simulink model "DCDC_PSFB_with_Mosfet_Converter"  (R2024b)
settings: Solver=ode23t  StartTime=0.0  StopTime=0.2  RelTol=1e-3
values from neighbouring files (symbols this model uses):
  fs = 140e3    (= 140000)    [PSFB_Calculation_Code.m]    (also in PSFB_DCDC_Conveter_Calculation.m)
  Pout = 5500    [PSFB_Calculation_Code.m]    (also in PSFB_DCDC_Conveter_Calculation.m)
  R_load = (Vout^2) / Pout    (= 116.363636364)    [PSFB_Calculation_Code.m]    (also in PSFB_DCDC_Conveter_Calculation.m = 0.104727272727)
  Ts = 1/fs    (= 7.14285714286e-06)    [PSFB_Calculation_Code.m]    (also in PSFB_DCDC_Conveter_Calculation.m)
  Vin = 24    [PSFB_Calculation_Code.m]    (also in PSFB_DCDC_Conveter_Calculation.m = 800)
  Vout = 800    [PSFB_Calculation_Code.m]    (also in PSFB_DCDC_Conveter_Calculation.m = 24; PSFB_Result_Plot_Code.m = Vout_sig.Data(:))
  Vout_max = 815    [PSFB_Calculation_Code.m]    (also in PSFB_DCDC_Conveter_Calculation.m = 25)
undefined symbols (not defined in the file or in its folder): C, L
libraries: spsMosfetLib x8, spsCurrentMeasurementLib x6, spsSeriesRLCBranchLib x6, spsDiodeLib x4, spsVoltageMeasurementLib x4, spsMeanLib x3, slpidlib x2, spsDCVoltageSourceLib x1, spsGroundLib x1, spsLinearTransformerLib x1, sps_lib x1
settings Model: Creator=SUDHAK1  LastModifiedBy=SUDHAK1

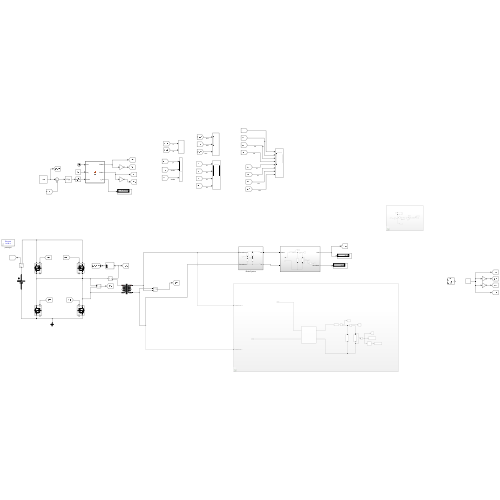
[thumbnail: Simulink's stored preview of the top-level diagram]
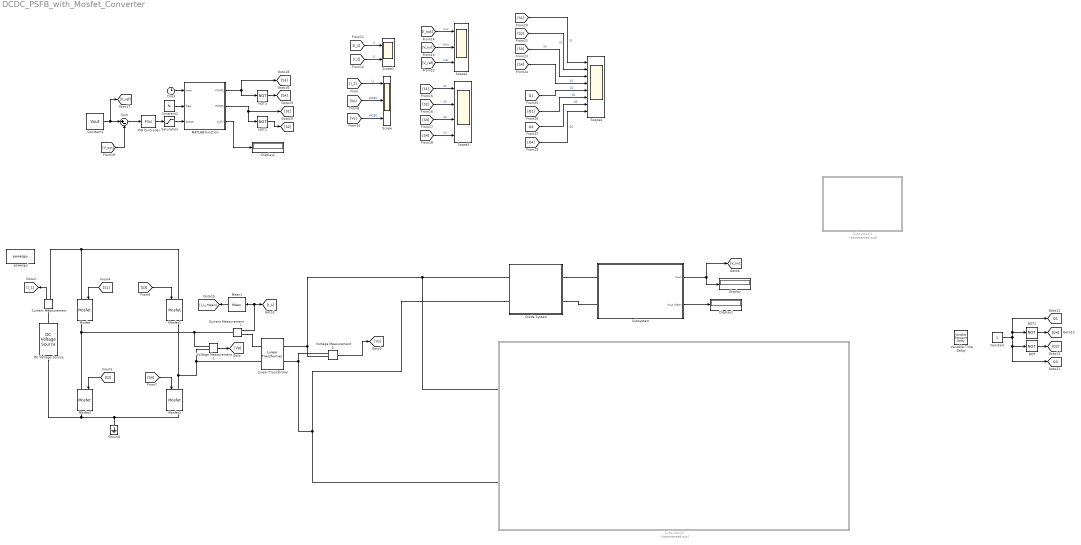
== system DCDC_PSFB_with_Mosfet_Converter ==
  Clock : Clock
  Constant : Constant
  Constant1 : Constant  Value=Vout
  Constant2 : Constant  Value=fs
  Current Measurement : spsCurrentMeasurementLib/Current Measurement  PhasorSimulation=off  OutputType=Complex  PSBequivalent=0
  Current Measurement1 : spsCurrentMeasurementLib/Current Measurement  PhasorSimulation=off  OutputType=Complex  PSBequivalent=0
  DC Voltage Source : spsDCVoltageSourceLib/DC Voltage Source  Amplitude=Vin  Measurements=None
  Diode System : Subsystem
  Display : Display
  Display1 : Display
  Display2 : Display
  Ground : spsGroundLib/Ground  LConnTagsString=a
  Linear Transformer : spsLinearTransformerLib/Linear Transformer  UNITS=SI  NominalPower=[Pout fs]  winding1=[Vin 4.3218e-9 0.45856e-9]  winding2=[Vout_max 0.7938e-9 0.084225e-9]  ThreeWindings=off  winding3=[Vout_max 0.7938e-9 0.084225e-9]  RmLm=[1.0804e+06 2866]  Measurements=None  DataType=on
  MATLAB Function : MATLAB Function  TreatAsAtomicUnit=on
  Mean1 : spsMeanLib/Mean  Freq=60  Vinit=0  Ts=0
  Mosfet{,1..3} (4 alike) : spsMosfetLib/Mosfet  Ron=0.1  Lon=0  Rd=0.01  Vfd=0  IC=0  Rs=1e5  Cs=inf  Measurements=on
  NOT{,1..3} (4 alike) : Logic  Operator=NOT  IconShape=distinctive  AllPortsSameDT=off  OutDataTypeStr=boolean
  PID Controller : slpidlib/PID Controller  Controller=PI  Form=Parallel  TimeDomain=Discrete-time  UseExternalTs=off  SampleTime=-1  IntegratorMethod=Forward Euler  FilterMethod=Forward Euler  ControllerParametersSource=internal  P=500  I=50  UseKiTs=off  D=0  UseExternalDerivativeSource=off  N=100  UseFilter=on  TunerSelectOption=Transfer Function Based (PID Tuner App)  InitialConditionSource=internal  InitialConditionForIntegrator=0  InitialConditionForFilter=0  DifferentiatorICPrevScaledInput=0  ExternalReset=none  TrackingMode=off  Kt=1  LimitOutput=off  SatLimitsSource=internal  UpperSaturationLimit=180  LowerSaturationLimit=0  LinearizeAsGain=on  AntiWindupMode=none  Kb=1  LimitIntegrator=off  UpperIntegratorSaturationLimit=inf  LowerIntegratorSaturationLimit=-inf  POutMin=[]  POutMax=[]  IOutMin=[]  IOutMax=[]  DOutMin=[]  DOutMax=[]  NOutMin=[]  NOutMax=[]  SumOutMin=[]  SumOutMax=[]  SaturationOutMin=[]  SaturationOutMax=[]  PParamMin=[]  PParamMax=[]  IParamMin=[]  IParamMax=[]  DParamMin=[]  DParamMax=[]  NParamMin=[]  NParamMax=[]  KbParamMin=[]  KbParamMax=[]  KtParamMin=[]  KtParamMax=[]  KbOutMin=[]  KbOutMax=[]  KtOutMin=[]  KtOutMax=[]  IntegratorOutMin=[]  IntegratorOutMax=[]  FilterOutMin=[]  FilterOutMax=[]  SumI1OutMin=[]  SumI1OutMax=[]  SumI2OutMin=[]  SumI2OutMax=[]  SumI3OutMin=[]  SumI3OutMax=[]  SumI4OutMin=[]  SumI4OutMax=[]  SumDOutMin=[]  SumDOutMax=[]  DifferentiatorOutMin=[]  DifferentiatorOutMax=[]  FilterDiffOutCoefMin=[]  FilterDiffOutCoefMax=[]  ReciprocalOutMin=[]  ReciprocalOutMax=[]  SumDenOutMin=[]  SumDenOutMax=[]  SumNumOutMin=[]  SumNumOutMax=[]  DivideOutMin=[]  DivideOutMax=[]  UdiffTsProdOutMin=[]  UdiffTsProdOutMax=[]  NTsProdOutMin=[]  NTsProdOutMax=[]  UintegralTsProdOutMin=[]  UintegralTsProdOutMax=[]  UngainTsProdOutMin=[]  UngainTsProdOutMax=[]  ClampingZeroOutDataTypeStr=Inherit: Inherit via back propagation  ClampingZeroOutMin=[]  ClampingZeroOutMax=[]  FilterDenConstantOutDataTypeStr=Inherit: Inherit via back propagation  FilterDenConstantOutMin=[]  FilterDenConstantOutMax=[]  PCopyOutDataTypeStr=Inherit: Inherit via back propagation  PCopyOutMin=[]  PCopyOutMax=[]  NCopyOutDataTypeStr=Inherit: Inherit via back propagation  NCopyOutMin=[]  NCopyOutMax=[]  IntegratorContinuousStateAttributes=''  IntegratorStateMustResolveToSignalObject=off  IntegratorRTWStateStorageClass=Auto  FilterContinuousStateAttributes=''  FilterStateMustResolveToSignalObject=off  FilterRTWStateStorageClass=Auto  ParallelPVariant=InternalParameters  IdealPVariant=Disabled  IVariant=InternalParameters  DVariant=Disabled  IntegratorVariant=Discrete  SatVariant=Disabled  AWVariant=Passthrough  PCopyVariant=Disabled  TRVariant=Disabled  FdbkBlocksVariant=Forward  IdealPFdbkVariant=Disabled  SatFdbkVariant=Disabled  DerivativeFilterVariant=Disabled  NVariant=Disabled  NCopyVariant=Disabled_SignalSpec  FilterICVariant=Disabled  IntegratorICVariant=InternalICs  ExternalResetVariant=Disabled  TRSumVariant=Passthrough  SumFdbkVariant=Disabled  SumVariant=Sum_PI  TsampFilterVariant=InternalTs  TsampNgainVariant=Passthrough  TsampIntegralVariant=Disabled_SignalSpec  ExternalSaturationOutDataTypeStr=Inherit: Same as second input  DerivativeSourceVariant=Disabled  PreIntVariant=InternalPreInt
  Saturation : Saturate  UpperLimit=180  LowerLimit=0
  Scope : Scope  NumInputPorts=3
  Scope1 : Scope  NumInputPorts=2
  Scope2 : Scope  NumInputPorts=3
  Scope3 : Scope  NumInputPorts=4
  Scope4 : Scope  NumInputPorts=8
  Subsystem : Subsystem
  Subsystem1 : Subsystem  Commented=on
  Subsystem2 : Subsystem  Commented=on
  Sum : Sum  Inputs=|+-
  Variable Time Delay : VariableTransportDelay  MaximumDelay=10
  Voltage Measurement1 : spsVoltageMeasurementLib/Voltage Measurement  PhasorSimulation=off  OutputType=Complex  PSBequivalent=0
  Voltage Measurement2 : spsVoltageMeasurementLib/Voltage Measurement  PhasorSimulation=off  OutputType=Complex  PSBequivalent=0
  powergui : sps_lib/powergui  Priority=1  SimulationMode=Discrete  SampleTime=Ts/1000  frequency=60  Iterations=50  frequencyindice=0  Pbase=100e6  ErrMax=1e-4  UnitsV=kV  UnitsW=MW  buscounter=0  FunctionMessages=off  echomessages=off  EnableUseOfTLC=off  CurrentSourceSwitches=off  DisableSnubberDevices=off  DisableRonSwitches=off  DisableVfSwitches=off  DisplayEquations=off  AutomaticDiscreteSolvers=off  SolverType=Tustin/Backward Euler (TBE)  Interpol=off  ExternalGateDelay=off  methode=off  Ts=100  x0status=blocks  SPID=on  SwTol=0  HookPort=off  NonlinearTolerance=1e-4  nMaxIteration=100  ContinueOnMaxIteration=off  RestoreLinks=warning  ResistiveCurrentMeasurement=off  Frange=[0:2:500]  Ylog=off  Xlog=on  ShowGrid=off  save=off  variable=ZData  structure=0  ZoomFFT=off  StartTime=0.0  cycles=1  DisplayStyle=1  fundamental=60  FreqAxis=off  MaxFrequency=1000  frequencyindicesteady=1  RmsSteady=1  display=off
  tag scope: Q1=global, Q3=global
  wires:
  [V_ref] -> Scope2/3  "Vref"
  Mean1/1 -> [I_L_mean]
  [S2] -> Mosfet2/1
  [I_2] -> Scope1/2  "I2"
  [V_out] -> Scope2/2  "Vout"
  [S2] -> Scope3/2  "S2"
  Current Measurement/1 -> [I_1]
  [I_2] -> Scope/1  "I_L"
  [S1] -> Mosfet/1
  [I_1] -> Scope1/1  "I1"
  [Vp] -> Scope/2  "VA1B1"
  [I_out] -> Scope2/1  "Iout"
  Voltage Measurement1/1 -> [Vp]
  Current Measurement1/1 -> Mean1/1, [I_L]
  Voltage Measurement2/1 -> [Vs]
  [S1] -> Scope3/1  "S1"
  [Vs] -> Scope/3  "VA2B2"
  [S4] -> Mosfet3/1
  [S3] -> Mosfet1/1
  [S3] -> Scope3/3  "S3"
  [S4] -> Scope3/4  "S4"
  [S1] -> Scope4/1  "S1"
  [S2] -> Scope4/2  "S2"
  [S4] -> Scope4/4  "S4"
  [S3] -> Scope4/3  "S3"
  [Q2] -> Scope4/6  "Q2"
  [Q1] -> Scope4/5  "Q1"
  [Q4] -> Scope4/8  "Q4"
  [Q3] -> Scope4/7  "Q3"
  Constant/1 -> [Q3], NOT/1, [Q1], NOT1/1
  Constant1/1 -> [V_ref], Sum/1
  MATLAB Function/3(t_phi) -> Display2/1
  NOT2/1 -> [S2]
  Sum/1 -> PID Controller/1
  Constant2/1 -> MATLAB Function/2(freq)
  Clock/1 -> MATLAB Function/1(time)
  PID Controller/1 -> Saturation/1
  [V_out] -> Sum/2
  MATLAB Function/1(PWM2) -> NOT3/1, [S3]
  MATLAB Function/2(PWM1) -> NOT2/1, [S1]
  Saturation/1 -> MATLAB Function/3(phase)
  NOT3/1 -> [S4]
  Subsystem/1(Vout) -> Display/1, [V_out]
  Subsystem/2(Vout Mean) -> Display1/1
  NOT/1 -> [Q2]
  NOT1/1 -> [Q4]
  connections:
  Mosfet2/RConn1 -- DC Voltage Source/LConn1 -- Ground/LConn1 -- Mosfet3/RConn1
  Mosfet1/RConn1 -- Voltage Measurement1/LConn2 -- Linear Transformer/LConn2 -- Mosfet3/LConn1
  Mosfet/LConn1 -- Current Measurement/RConn1 -- Mosfet1/LConn1
  DC Voltage Source/RConn1 -- Current Measurement/LConn1
  Current Measurement1/RConn1 -- Linear Transformer/LConn1
  Diode System/LConn1 -- Subsystem2/LConn1 -- Voltage Measurement2/LConn1 -- Linear Transformer/RConn1
  Diode System/LConn2 -- Subsystem2/LConn2 -- Voltage Measurement2/LConn2 -- Linear Transformer/RConn2
  Diode System/RConn1 -- Subsystem/LConn1
  Diode System/RConn2 -- Subsystem/LConn2
  Mosfet/RConn1 -- Current Measurement1/LConn1 -- Voltage Measurement1/LConn1 -- Mosfet2/LConn1

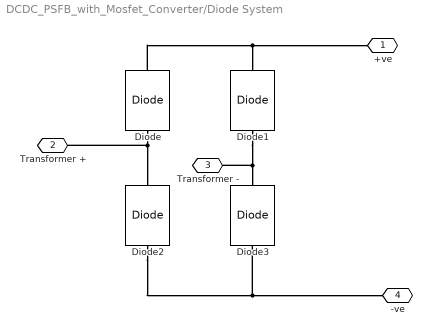
== system DCDC_PSFB_with_Mosfet_Converter/Diode System ==
  Diode{,1..3} (4 alike) : spsDiodeLib/Diode  Ron=0.001  Lon=0  Vf=0.8  IC=0  UseSnubber=0  Rs=500  Cs=250e-9  Measurements=off
  +ve : PMIOPort  Side=Right
  Transformer + : PMIOPort  Port=2  Side=Left
  Transformer - : PMIOPort  Port=3  Side=Left
  -ve : PMIOPort  Port=4  Side=Right
  connections:
  Diode/RConn1 -- Diode1/RConn1 -- +ve/RConn1
  Diode/LConn1 -- Transformer +/RConn1 -- Diode2/RConn1
  Diode2/LConn1 -- Diode3/LConn1 -- -ve/RConn1
  Diode1/LConn1 -- Diode3/RConn1 -- Transformer -/RConn1

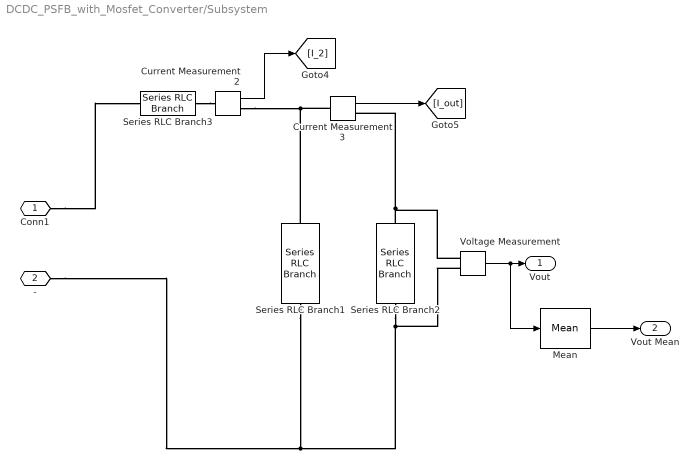
== system DCDC_PSFB_with_Mosfet_Converter/Subsystem ==
  Current Measurement2 : spsCurrentMeasurementLib/Current Measurement  PhasorSimulation=off  OutputType=Complex  PSBequivalent=0
  Current Measurement3 : spsCurrentMeasurementLib/Current Measurement  PhasorSimulation=off  OutputType=Complex  PSBequivalent=0
  Mean : spsMeanLib/Mean  Freq=60  Vinit=0  Ts=0
  Series RLC Branch1 : spsSeriesRLCBranchLib/Series RLC Branch  LConnTagsString=__new0  RConnTagsString=__new0  BranchType=C  Resistance=1  Inductance=7.8e-7  SetiL0=off  InitialCurrent=0  Capacitance=C*2.5  Setx0=off  InitialVoltage=0  Measurements=None
  Series RLC Branch2 : spsSeriesRLCBranchLib/Series RLC Branch  LConnTagsString=__new0  RConnTagsString=__new0  BranchType=R  Resistance=R_load  Inductance=1e-3  SetiL0=off  InitialCurrent=0  Capacitance=1e-6  Setx0=off  InitialVoltage=0  Measurements=None
  Series RLC Branch3 : spsSeriesRLCBranchLib/Series RLC Branch  LConnTagsString=__new0  RConnTagsString=__new0  BranchType=L  Resistance=1  Inductance=L  SetiL0=off  InitialCurrent=0  Capacitance=1e-6  Setx0=off  InitialVoltage=0  Measurements=None
  Voltage Measurement : spsVoltageMeasurementLib/Voltage Measurement  PhasorSimulation=off  OutputType=Complex  PSBequivalent=0
  Conn1 : PMIOPort  Side=Left
  - : PMIOPort  Port=2  Side=Left
  Vout : Outport
  Vout Mean : Outport  Port=2
  wires:
  Current Measurement3/1 -> [I_out]
  Current Measurement2/1 -> [I_2]
  Mean/1 -> Vout Mean/1
  Voltage Measurement/1 -> Mean/1, Vout/1
  connections:
  Series RLC Branch2/LConn1 -- Current Measurement3/RConn1 -- Voltage Measurement/LConn1
  Voltage Measurement/LConn2 -- -/RConn1 -- Series RLC Branch1/RConn1 -- Series RLC Branch2/RConn1
  Series RLC Branch3/RConn1 -- Current Measurement2/LConn1
  Series RLC Branch1/LConn1 -- Current Measurement2/RConn1 -- Current Measurement3/LConn1
  Conn1/RConn1 -- Series RLC Branch3/LConn1

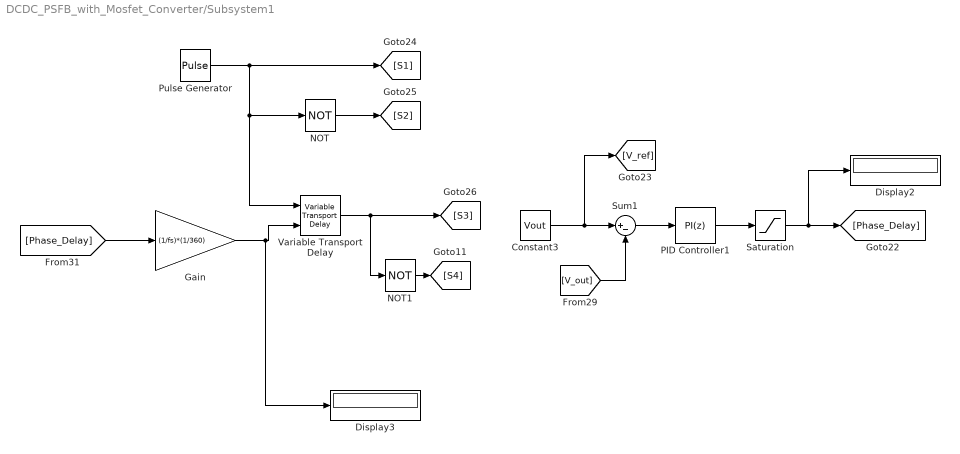
== system DCDC_PSFB_with_Mosfet_Converter/Subsystem1 ==
  Constant3 : Constant  Value=Vout
  Display2 : Display
  Display3 : Display
  Gain : Gain  Gain=(1/fs)*(1/360)
  NOT : Logic  Operator=NOT  IconShape=distinctive  AllPortsSameDT=off  OutDataTypeStr=boolean
  NOT1 : Logic  Operator=NOT  IconShape=distinctive  AllPortsSameDT=off  OutDataTypeStr=boolean
  PID Controller1 : slpidlib/PID Controller  Controller=PI  Form=Parallel  TimeDomain=Discrete-time  UseExternalTs=off  SampleTime=-1  IntegratorMethod=Forward Euler  FilterMethod=Forward Euler  ControllerParametersSource=internal  P=50000  I=500  UseKiTs=off  D=0  UseExternalDerivativeSource=off  N=100  UseFilter=on  TunerSelectOption=Transfer Function Based (PID Tuner App)  InitialConditionSource=internal  InitialConditionForIntegrator=0  InitialConditionForFilter=0  DifferentiatorICPrevScaledInput=0  ExternalReset=none  TrackingMode=off  Kt=1  LimitOutput=off  SatLimitsSource=internal  UpperSaturationLimit=inf  LowerSaturationLimit=-inf  LinearizeAsGain=on  AntiWindupMode=none  Kb=1  LimitIntegrator=off  UpperIntegratorSaturationLimit=inf  LowerIntegratorSaturationLimit=-inf  POutMin=[]  POutMax=[]  IOutMin=[]  IOutMax=[]  DOutMin=[]  DOutMax=[]  NOutMin=[]  NOutMax=[]  SumOutMin=[]  SumOutMax=[]  SaturationOutMin=[]  SaturationOutMax=[]  PParamMin=[]  PParamMax=[]  IParamMin=[]  IParamMax=[]  DParamMin=[]  DParamMax=[]  NParamMin=[]  NParamMax=[]  KbParamMin=[]  KbParamMax=[]  KtParamMin=[]  KtParamMax=[]  KbOutMin=[]  KbOutMax=[]  KtOutMin=[]  KtOutMax=[]  IntegratorOutMin=[]  IntegratorOutMax=[]  FilterOutMin=[]  FilterOutMax=[]  SumI1OutMin=[]  SumI1OutMax=[]  SumI2OutMin=[]  SumI2OutMax=[]  SumI3OutMin=[]  SumI3OutMax=[]  SumI4OutMin=[]  SumI4OutMax=[]  SumDOutMin=[]  SumDOutMax=[]  DifferentiatorOutMin=[]  DifferentiatorOutMax=[]  FilterDiffOutCoefMin=[]  FilterDiffOutCoefMax=[]  ReciprocalOutMin=[]  ReciprocalOutMax=[]  SumDenOutMin=[]  SumDenOutMax=[]  SumNumOutMin=[]  SumNumOutMax=[]  DivideOutMin=[]  DivideOutMax=[]  UdiffTsProdOutMin=[]  UdiffTsProdOutMax=[]  NTsProdOutMin=[]  NTsProdOutMax=[]  UintegralTsProdOutMin=[]  UintegralTsProdOutMax=[]  UngainTsProdOutMin=[]  UngainTsProdOutMax=[]  ClampingZeroOutDataTypeStr=Inherit: Inherit via back propagation  ClampingZeroOutMin=[]  ClampingZeroOutMax=[]  FilterDenConstantOutDataTypeStr=Inherit: Inherit via back propagation  FilterDenConstantOutMin=[]  FilterDenConstantOutMax=[]  PCopyOutDataTypeStr=Inherit: Inherit via back propagation  PCopyOutMin=[]  PCopyOutMax=[]  NCopyOutDataTypeStr=Inherit: Inherit via back propagation  NCopyOutMin=[]  NCopyOutMax=[]  IntegratorContinuousStateAttributes=''  IntegratorStateMustResolveToSignalObject=off  IntegratorRTWStateStorageClass=Auto  FilterContinuousStateAttributes=''  FilterStateMustResolveToSignalObject=off  FilterRTWStateStorageClass=Auto  ParallelPVariant=InternalParameters  IdealPVariant=Disabled  IVariant=InternalParameters  DVariant=Disabled  IntegratorVariant=Discrete  SatVariant=Disabled  AWVariant=Passthrough  PCopyVariant=Disabled  TRVariant=Disabled  FdbkBlocksVariant=Forward  IdealPFdbkVariant=Disabled  SatFdbkVariant=Disabled  DerivativeFilterVariant=Disabled  NVariant=Disabled  NCopyVariant=Disabled_SignalSpec  FilterICVariant=Disabled  IntegratorICVariant=InternalICs  ExternalResetVariant=Disabled  TRSumVariant=Passthrough  SumFdbkVariant=Disabled  SumVariant=Sum_PI  TsampFilterVariant=InternalTs  TsampNgainVariant=Passthrough  TsampIntegralVariant=Disabled_SignalSpec  ExternalSaturationOutDataTypeStr=Inherit: Same as second input  DerivativeSourceVariant=Disabled  PreIntVariant=InternalPreInt
  Pulse Generator : DiscretePulseGenerator  PulseType=Time based  Period=1/fs  PulseWidth=50
  Saturation : Saturate  UpperLimit=180  LowerLimit=0
  Sum1 : Sum  Inputs=|+-
  Variable Transport Delay : VariableTransportDelay  MaximumDelay=10
  wires:
  [V_out] -> Sum1/2
  Gain/1 -> Display3/1, Variable Transport Delay/2
  NOT1/1 -> [S4]
  PID Controller1/1 -> Saturation/1
  Constant3/1 -> [V_ref], Sum1/1
  Saturation/1 -> Display2/1, [Phase_Delay]
  Sum1/1 -> PID Controller1/1
  [Phase_Delay] -> Gain/1
  Variable Transport Delay/1 -> NOT1/1, [S3]
  Pulse Generator/1 -> Variable Transport Delay/1, NOT/1, [S1]
  NOT/1 -> [S2]

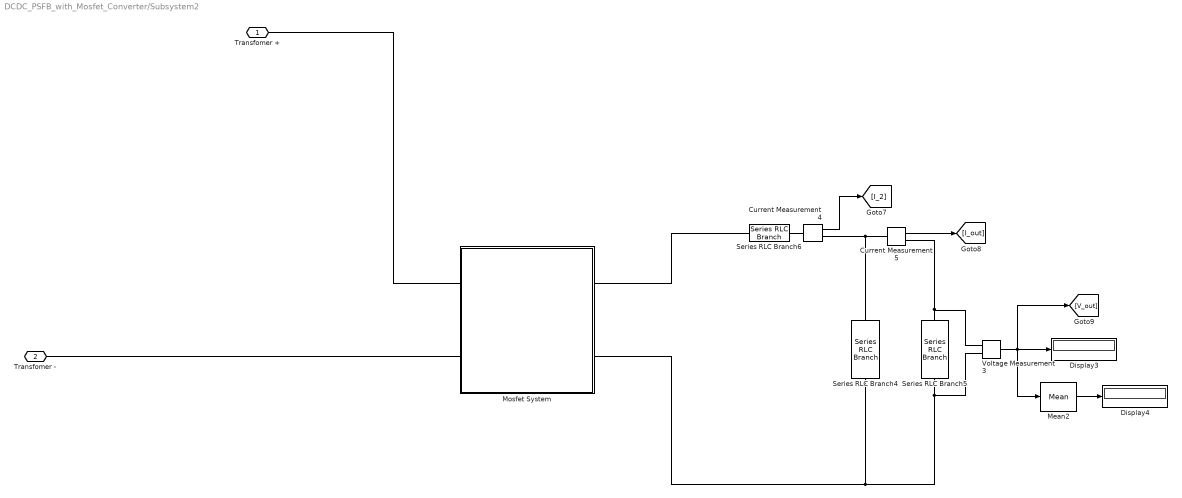
== system DCDC_PSFB_with_Mosfet_Converter/Subsystem2 ==
  Current Measurement4 : spsCurrentMeasurementLib/Current Measurement  PhasorSimulation=off  OutputType=Complex  PSBequivalent=0
  Current Measurement5 : spsCurrentMeasurementLib/Current Measurement  PhasorSimulation=off  OutputType=Complex  PSBequivalent=0
  Display3 : Display
  Display4 : Display
  Mean2 : spsMeanLib/Mean  Freq=60  Vinit=0  Ts=0
  Mosfet System : Subsystem
  Series RLC Branch4 : spsSeriesRLCBranchLib/Series RLC Branch  LConnTagsString=__new0  RConnTagsString=__new0  BranchType=C  Resistance=1  Inductance=7.8e-7  SetiL0=off  InitialCurrent=0  Capacitance=C*2.5  Setx0=off  InitialVoltage=0  Measurements=None
  Series RLC Branch5 : spsSeriesRLCBranchLib/Series RLC Branch  LConnTagsString=__new0  RConnTagsString=__new0  BranchType=R  Resistance=R_load  Inductance=1e-3  SetiL0=off  InitialCurrent=0  Capacitance=1e-6  Setx0=off  InitialVoltage=0  Measurements=None
  Series RLC Branch6 : spsSeriesRLCBranchLib/Series RLC Branch  LConnTagsString=__new0  RConnTagsString=__new0  BranchType=L  Resistance=1  Inductance=L  SetiL0=off  InitialCurrent=0  Capacitance=1e-6  Setx0=off  InitialVoltage=0  Measurements=None
  Voltage Measurement3 : spsVoltageMeasurementLib/Voltage Measurement  PhasorSimulation=off  OutputType=Complex  PSBequivalent=0
  Transfomer + : PMIOPort  Side=Left
  Transfomer - : PMIOPort  Port=2  Side=Left
  wires:
  Current Measurement4/1 -> [I_2]
  Current Measurement5/1 -> [I_out]
  Voltage Measurement3/1 -> Display3/1, [V_out], Mean2/1
  Mean2/1 -> Display4/1
  connections:
  Series RLC Branch5/RConn1 -- Mosfet System/RConn2 -- Series RLC Branch4/RConn1 -- Voltage Measurement3/LConn2
  Voltage Measurement3/LConn1 -- Series RLC Branch5/LConn1 -- Current Measurement5/RConn1
  Series RLC Branch6/LConn1 -- Mosfet System/RConn1
  Series RLC Branch6/RConn1 -- Current Measurement4/LConn1
  Series RLC Branch4/LConn1 -- Current Measurement4/RConn1 -- Current Measurement5/LConn1
  Mosfet System/LConn2 -- Transfomer -/RConn1
  Mosfet System/LConn1 -- Transfomer +/RConn1

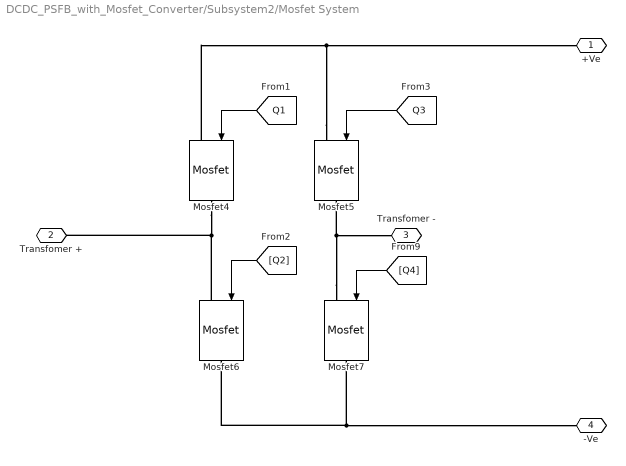
== system DCDC_PSFB_with_Mosfet_Converter/Subsystem2/Mosfet System ==
  Mosfet{4..7} (4 alike) : spsMosfetLib/Mosfet  Ron=0.1  Lon=0  Rd=0.01  Vfd=0  IC=0  Rs=1e5  Cs=inf  Measurements=off
  +Ve : PMIOPort  Side=Right
  Transfomer + : PMIOPort  Port=2  Side=Left
  Transfomer - : PMIOPort  Port=3  Side=Left
  -Ve : PMIOPort  Port=4  Side=Right
  wires:
  [Q1] -> Mosfet4/1
  [Q3] -> Mosfet5/1
  [Q4] -> Mosfet7/1
  [Q2] -> Mosfet6/1
  connections:
  Mosfet4/RConn1 -- Transfomer +/RConn1 -- Mosfet6/LConn1
  Mosfet7/RConn1 -- Mosfet6/RConn1 -- -Ve/RConn1
  Mosfet5/LConn1 -- +Ve/RConn1 -- Mosfet4/LConn1
  Mosfet7/LConn1 -- Transfomer -/RConn1 -- Mosfet5/RConn1

== matlab function DCDC_PSFB_with_Mosfet_Converter/MATLAB Function ==
  data: time input; PWM2 output; PWM1 output; freq input; phase input; t_phi output
function [PWM2,PWM1,t_phi] = fcn(time,freq,phase)
Tswitching = 1/freq;
PWM1 = 0;
PWM2 = 0;

y1 = mod(time,Tswitching);

if y1 < Tswitching/2
    PWM1 = 1;
end 

t_phi = Tswitching*phase/360;

y2=mod(time+t_phi,Tswitching);

if y2 < Tswitching/2
    PWM2 = 1;
end
